simulink model "ACC5v_FFNN_traincgf_30_30_30_ep_50_Nor_20250704"  (R2021a)
settings: Solver=FixedStepAuto  StartTime=0.0  StopTime=T  RelTol=1e-3
undefined symbols (not defined in the file or in its folder): t_gap, Ts, v0_ego, v0_lead, v_set, x0_ego, x0_lead, x_gain, x_offset, y_gain, y_offset
libraries: neural x95
(part 1 of 5)
settings Model: Creator=The MathWorks, Inc.  LastModifiedBy=deyun
settings SolverCC: AlgebraicLoopSolver=TrustRegion
settings DataIOCC: ReturnWorkspaceOutputs=off
settings DebuggingCC: ArithmeticOperatorsInVariantConditions=warning
settings SFSimCC: SimUseLocalCustomCode=off  CustomCodeUndefinedFunction=UseInterfaceOnly
settings RTWCC: RTWUseLocalCustomCode=off
settings CodeAppCC: StateflowObjectComments=on

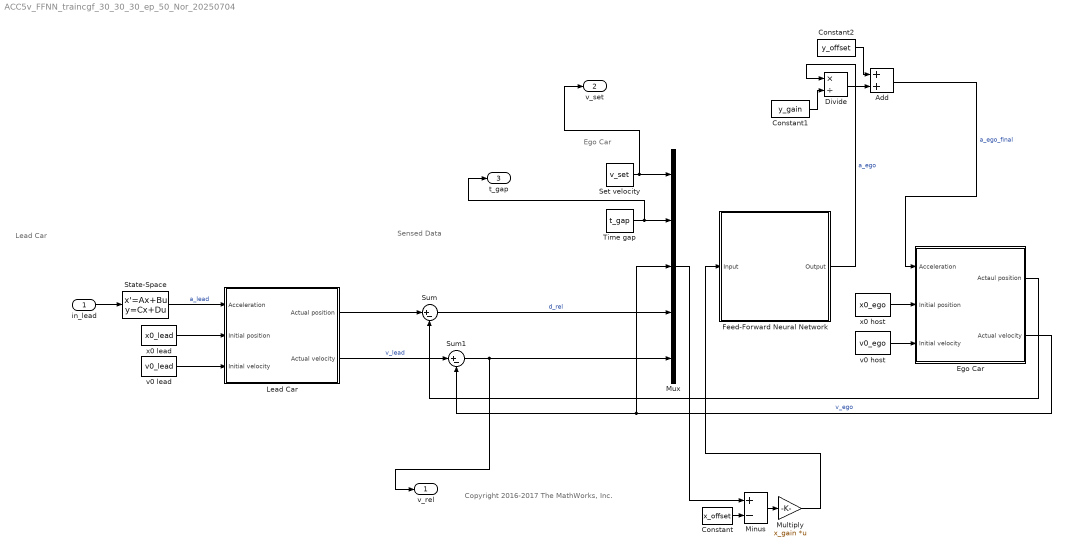
== system ACC5v_FFNN_traincgf_30_30_30_ep_50_Nor_20250704 ==
  note: Sensed Data
  note: Lead Car
  note: Ego Car
  note: Copyright 2016-2017 The MathWorks, Inc.
  in_lead : Inport
  Add : Sum
  Constant : Constant  Value=x_offset
  Constant1 : Constant  Value=y_gain
  Constant2 : Constant  Value=y_offset
  Divide : Product  Inputs=*/
  Ego Car : Subsystem
  Feed-Forward Neural Network : Subsystem
      mask help: Feed-Forward Neural Network
      mask Display: e = 0.06;c1 = [120 150 230]/255;c2 = ([120 150 230]+0)/383;c3 = ([120 150 230]+128)/383;patch([0 1 1 0],[0 0 1 1],c1);patch([0 1 1 1-e 1-e 0+e],[0 0 1 1-e 0+e 0+e],c2);patch([0 0 1 1-e 0+e 0+e],[0 1 1 1-e 1-e 0+e],c3);plot([0 1 1 0 0],[0 0 1 1 0]);fprintf('NNET');port_label('input',1,' Input');port_label('output',1,'Output ');
  Lead Car : Subsystem
  Minus : Sum  Inputs=+-
  Multiply : Gain  Gain=x_gain  Multiplication=Matrix(K*u)
  Mux : Mux  Inputs=5
  Set velocity : Constant  Value=v_set  SampleTime=Ts
  State-Space : StateSpace  A=-10  B=10  D=0  InitialCondition=0
  Sum : Sum  Inputs=|+-
  Sum1 : Sum  Inputs=|+-
  Time gap : Constant  Value=t_gap  SampleTime=Ts
  v0 host : Constant  Value=v0_ego  SampleTime=Ts
  v0 lead : Constant  Value=v0_lead  SampleTime=Ts
  x0 host : Constant  Value=x0_ego  SampleTime=Ts
  x0 lead : Constant  Value=x0_lead  SampleTime=Ts
  v_rel : Outport
  v_set : Outport  Port=2
  t_gap : Outport  Port=3
  wires:
  x0 lead/1 -> Lead Car/2(Initial position)
  v0 lead/1 -> Lead Car/3(Initial velocity)
  x0 host/1 -> Ego Car/2(Initial position)
  Ego Car/1(Actaul position) -> Sum/2
  Ego Car/2(Actual velocity) -> Mux/3, Sum1/2  "v_ego"
  v0 host/1 -> Ego Car/3(Initial velocity)
  Set velocity/1 -> v_set/1, Mux/1
  Feed-Forward Neural Network/1(Output) -> Divide/1  "a_ego"
  Lead Car/1(Actual position) -> Sum/1
  Sum1/1 -> v_rel/1, Mux/5
  State-Space/1 -> Lead Car/1(Acceleration)  "a_lead"
  Lead Car/2(Actual velocity) -> Sum1/1  "v_lead"
  Sum/1 -> Mux/4  "d_rel"
  in_lead/1 -> State-Space/1
  Time gap/1 -> t_gap/1, Mux/2
  Mux/1 -> Minus/1
  Minus/1 -> Multiply/1
  Constant/1 -> Minus/2
  Multiply/1 -> Feed-Forward Neural Network/1(Input)
  Constant1/1 -> Divide/2
  Divide/1 -> Add/2
  Constant2/1 -> Add/1
  Add/1 -> Ego Car/1(Acceleration)  "a_ego_final"

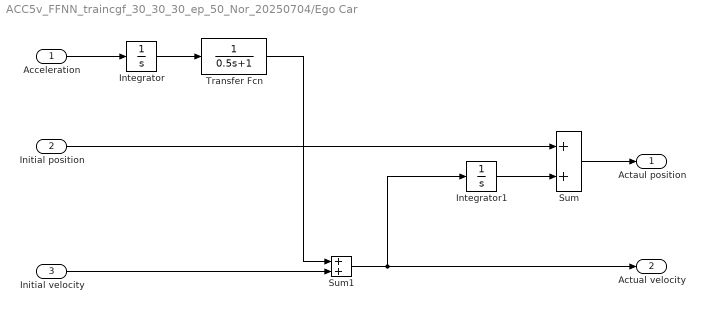
== system ACC5v_FFNN_traincgf_30_30_30_ep_50_Nor_20250704/Ego Car ==
  Acceleration : Inport
  Initial position : Inport  Port=2
  Initial velocity : Inport  Port=3
  Integrator : Integrator
  Integrator1 : Integrator
  Sum : Sum
  Sum1 : Sum
  Transfer Fcn : TransferFcn  Denominator=[0.5 1]
  Actaul position : Outport  VectorParamsAs1DForOutWhenUnconnected=off
  Actual velocity : Outport  Port=2  VectorParamsAs1DForOutWhenUnconnected=off
  wires:
  Sum1/1 -> Integrator1/1, Actual velocity/1
  Initial velocity/1 -> Sum1/2
  Sum/1 -> Actaul position/1
  Transfer Fcn/1 -> Sum1/1
  Integrator/1 -> Transfer Fcn/1
  Acceleration/1 -> Integrator/1
  Initial position/1 -> Sum/1
  Integrator1/1 -> Sum/2

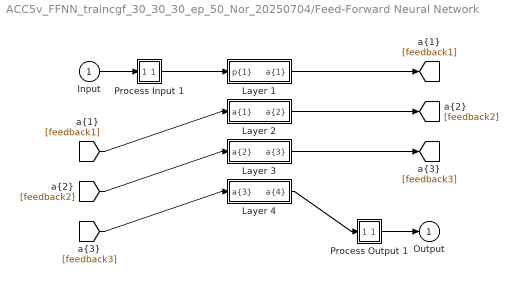
== system ACC5v_FFNN_traincgf_30_30_30_ep_50_Nor_20250704/Feed-Forward Neural Network ==
  Input : Inport  PortDimensions=5
      mask Display: e = 0.06;c1 = [120 230 180]/255;c2 = ([120 230 180]+0)/(256+128);c3 = ([120 230 180]+128)/(256+128);patch([0 1 1 0],[0 0 1 1],c1);patch([0 1 1 1-e 1-e 0+e],[0 0 1 1-e 0+e 0+e],c2);patch([0 0 1 1-e 0+e 0+e],[0 1 1 1-e 1-e 0+e],c3);plot([0 1 1 0 0],[0 0 1 1 0]);
  Layer 1 : Subsystem
      mask Display: e = 0.06;c1 = [120 150 230]/255;c2 = ([120 150 230]+0)/383;c3 = ([120 150 230]+128)/383;patch([0 1 1 0],[0 0 1 1],c1);patch([0 1 1 1-e 1-e 0+e],[0 0 1 1-e 0+e 0+e],c2);patch([0 0 1 1-e 0+e 0+e],[0 1 1 1-e 1-e 0+e],c3);plot([0 1 1 0 0],[0 0 1 1 0]);
  Layer 2 : Subsystem
      mask Display: e = 0.06;c1 = [120 150 230]/255;c2 = ([120 150 230]+0)/383;c3 = ([120 150 230]+128)/383;patch([0 1 1 0],[0 0 1 1],c1);patch([0 1 1 1-e 1-e 0+e],[0 0 1 1-e 0+e 0+e],c2);patch([0 0 1 1-e 0+e 0+e],[0 1 1 1-e 1-e 0+e],c3);plot([0 1 1 0 0],[0 0 1 1 0]);
  Layer 3 : Subsystem
      mask Display: e = 0.06;c1 = [120 150 230]/255;c2 = ([120 150 230]+0)/383;c3 = ([120 150 230]+128)/383;patch([0 1 1 0],[0 0 1 1],c1);patch([0 1 1 1-e 1-e 0+e],[0 0 1 1-e 0+e 0+e],c2);patch([0 0 1 1-e 0+e 0+e],[0 1 1 1-e 1-e 0+e],c3);plot([0 1 1 0 0],[0 0 1 1 0]);
  Layer 4 : Subsystem
      mask Display: e = 0.06;c1 = [120 150 230]/255;c2 = ([120 150 230]+0)/383;c3 = ([120 150 230]+128)/383;patch([0 1 1 0],[0 0 1 1],c1);patch([0 1 1 1-e 1-e 0+e],[0 0 1 1-e 0+e 0+e],c2);patch([0 0 1 1-e 0+e 0+e],[0 1 1 1-e 1-e 0+e],c3);plot([0 1 1 0 0],[0 0 1 1 0]);
  Process Input 1 : Subsystem
      mask Display: e = 0.06;c1 = [120 150 230]/255;c2 = ([120 150 230]+0)/383;c3 = ([120 150 230]+128)/383;patch([0 1 1 0],[0 0 1 1],c1);patch([0 1 1 1-e 1-e 0+e],[0 0 1 1-e 0+e 0+e],c2);patch([0 0 1 1-e 0+e 0+e],[0 1 1 1-e 1-e 0+e],c3);plot([0 1 1 0 0],[0 0 1 1 0]);
  Process Output 1 : Subsystem
      mask Display: e = 0.06;c1 = [120 150 230]/255;c2 = ([120 150 230]+0)/383;c3 = ([120 150 230]+128)/383;patch([0 1 1 0],[0 0 1 1],c1);patch([0 1 1 1-e 1-e 0+e],[0 0 1 1-e 0+e 0+e],c2);patch([0 0 1 1-e 0+e 0+e],[0 1 1 1-e 1-e 0+e],c3);plot([0 1 1 0 0],[0 0 1 1 0]);
  Output : Outport  InitialOutput=0
      mask Display: e = 0.06;c1 = [120 230 180]/255;c2 = ([120 230 180]+0)/(256+128);c3 = ([120 230 180]+128)/(256+128);patch([0 1 1 0],[0 0 1 1],c1);patch([0 1 1 1-e 1-e 0+e],[0 0 1 1-e 0+e 0+e],c2);patch([0 0 1 1-e 0+e 0+e],[0 1 1 1-e 1-e 0+e],c3);plot([0 1 1 0 0],[0 0 1 1 0]);
  wires:
  Layer 4/1("a{4}") -> Process Output 1/1(a)
  [feedback3] -> Layer 4/1("a{3} ")
  Layer 3/1("a{3}") -> [feedback3]
  [feedback2] -> Layer 3/1("a{2} ")
  Layer 2/1("a{2}") -> [feedback2]
  [feedback1] -> Layer 2/1("a{1} ")
  Layer 1/1("a{1}") -> [feedback1]
  Process Input 1/1(p) -> Layer 1/1("p{1}")
  Process Output 1/1(y) -> Output/1
  Input/1 -> Process Input 1/1(x)

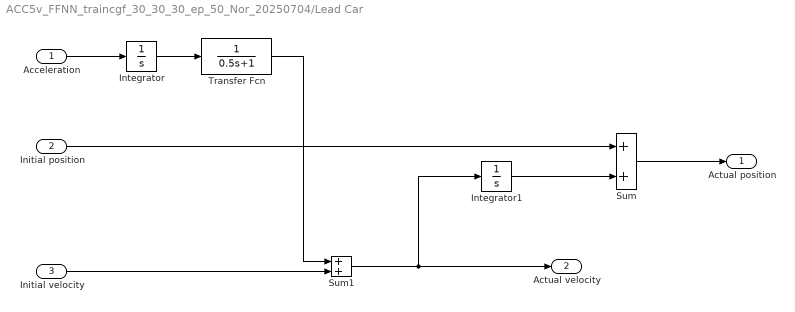
== system ACC5v_FFNN_traincgf_30_30_30_ep_50_Nor_20250704/Lead Car ==
  Acceleration : Inport
  Initial position : Inport  Port=2
  Initial velocity : Inport  Port=3
  Integrator : Integrator
  Integrator1 : Integrator
  Sum : Sum
  Sum1 : Sum
  Transfer Fcn : TransferFcn  Denominator=[0.5 1]
  Actual position : Outport  VectorParamsAs1DForOutWhenUnconnected=off
  Actual velocity : Outport  Port=2  VectorParamsAs1DForOutWhenUnconnected=off
  wires:
  Transfer Fcn/1 -> Sum1/1
  Initial velocity/1 -> Sum1/2
  Sum/1 -> Actual position/1
  Integrator/1 -> Transfer Fcn/1
  Sum1/1 -> Integrator1/1, Actual velocity/1
  Acceleration/1 -> Integrator/1
  Initial position/1 -> Sum/1
  Integrator1/1 -> Sum/2

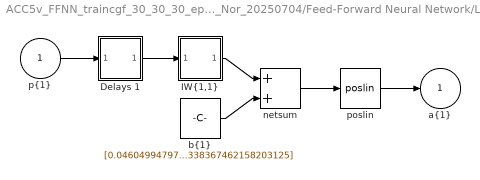
== system ACC5v_FFNN_traincgf_30_30_30_ep_50_Nor_20250704/Feed-Forward Neural Network/Layer 1 ==
  "p{1}" : Inport  PortDimensions=5
      mask Display: e = 0.06;c1 = [120 230 180]/255;c2 = ([120 230 180]+0)/(256+128);c3 = ([120 230 180]+128)/(256+128);patch([0 1 1 0],[0 0 1 1],c1);patch([0 1 1 1-e 1-e 0+e],[0 0 1 1-e 0+e 0+e],c2);patch([0 0 1 1-e 0+e 0+e],[0 1 1 1-e 1-e 0+e],c3);plot([0 1 1 0 0],[0 0 1 1 0]);
  Delays 1 : Subsystem
      mask Display: e = 0.06;c1 = [120 150 230]/255;c2 = ([120 150 230]+0)/383;c3 = ([120 150 230]+128)/383;patch([0 1 1 0],[0 0 1 1],c1);patch([0 1 1 1-e 1-e 0+e],[0 0 1 1-e 0+e 0+e],c2);patch([0 0 1 1-e 0+e 0+e],[0 1 1 1-e 1-e 0+e],c3);plot([0 1 1 0 0],[0 0 1 1 0]);disp('0');
  "IW{1,1}" : Subsystem
      mask Display: e = 0.06;c1 = [120 150 230]/255;c2 = ([120 150 230]+0)/383;c3 = ([120 150 230]+128)/383;patch([0 1 1 0],[0 0 1 1],c1);patch([0 1 1 1-e 1-e 0+e],[0 0 1 1-e 0+e 0+e],c2);patch([0 0 1 1-e 0+e 0+e],[0 1 1 1-e 1-e 0+e],c3);plot([0 1 1 0 0],[0 0 1 1 0]);disp('W');
  "b{1}" : Constant  Value=[0.0460499479730639149632764883790514431893825531005859375;-0.349402015011147870637842061114497482776641845703125;0.66507025600709568369239832463790662586688995361328125;0.60741250780027267186511608088039793074131011962890625;0.126284847005241951389820087570114992558956146240234375;-0.4740719325396856032028836125391535460948944091796875;0.3611324046089003925175120457424782216548919677734375;-0.5319955567783940519888119524694047868251800537109375;-0.08710031213979936570712681032091495580971240997314453125;-0.230866210976952146438634372316300868988037109375;0.077202877396043589897089987061917781829833984375;1.0025558120245303683759630075655877590179443359375;0.497318027802917728141807174324640072882175445556640625;0.9553277572718903432047454771236516535282135009765625;-0.496332469052459479552652510392363183200359344482421875;0.045748943680550525903161229734905646182596683502197265625;-0.897127892866184328823919713613577187061309814453125;0.5137509419692445344907127946498803794384002685546875;0.20395953255102039491930554504506289958953857421875;0.708157197743781718912714495672844350337982177734375;0.9532103730466758850781161527265794575214385986328125;0.85600360045154000321332432577037252485752105712890625;-0.165015832658127525878200003717211075127124786376953125;-1.004030844730705585021723891259171068668365478515625;0.0873034903187444033534347909153439104557037353515625;-0.5845387560078811883812477390165440738201141357421875;-0.5614328236351393552894251115503720939159393310546875;-0.3537174892029881778654498702962882816791534423828125;-0.80810116678483101537722177454270422458648681640625;0.4950673234766060915035268408246338367462158203125]
      mask Display: e = 0.06;c1 = [120 150 230]/255;c2 = ([120 150 230]+0)/383;c3 = ([120 150 230]+128)/383;patch([0 1 1 0],[0 0 1 1],c1);patch([0 1 1 1-e 1-e 0+e],[0 0 1 1-e 0+e 0+e],c2);patch([0 0 1 1-e 0+e 0+e],[0 1 1 1-e 1-e 0+e],c3);plot([0 1 1 0 0],[0 0 1 1 0]);disp('b');
  netsum : Sum  Inputs=2  InputSameDT=on  SaturateOnIntegerOverflow=on  OutDataTypeStr=Inherit: Same as first input
      mask Display: e = 0.06;c1 = [120 150 230]/255;c2 = ([120 150 230]+0)/383;c3 = ([120 150 230]+128)/383;patch([0 1 1 0],[0 0 1 1],c1);patch([0 1 1 1-e 1-e 0+e],[0 0 1 1-e 0+e 0+e],c2);patch([0 0 1 1-e 0+e 0+e],[0 1 1 1-e 1-e 0+e],c3);plot([0 1 1 0 0],[0 0 1 1 0]);disp('+');
  poslin : neural/Transfer Functions/poslin
      settings: SourceProductBaseCode=NN
  "a{1}" : Outport  InitialOutput=[0;0;0;0;0;0;0;0;0;0;0;0;0;0;0;0;0;0;0;0;0;0;0;0;0;0;0;0;0;0]
      mask Display: e = 0.06;c1 = [120 230 180]/255;c2 = ([120 230 180]+0)/(256+128);c3 = ([120 230 180]+128)/(256+128);patch([0 1 1 0],[0 0 1 1],c1);patch([0 1 1 1-e 1-e 0+e],[0 0 1 1-e 0+e 0+e],c2);patch([0 0 1 1-e 0+e 0+e],[0 1 1 1-e 1-e 0+e],c3);plot([0 1 1 0 0],[0 0 1 1 0]);
  wires:
  poslin/1 -> "a{1}"/1
  netsum/1 -> poslin/1
  "b{1}"/1 -> netsum/2
  "IW{1,1}"/1("iz{1,1}") -> netsum/1
  Delays 1/1("pd{1,1}") -> "IW{1,1}"/1("pd{1,1}")
  "p{1}"/1 -> Delays 1/1("p{1}")

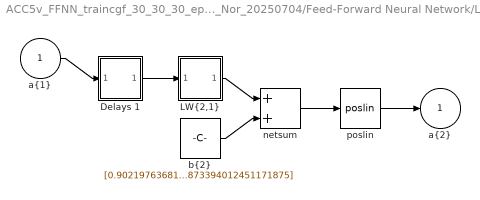
== system ACC5v_FFNN_traincgf_30_30_30_ep_50_Nor_20250704/Feed-Forward Neural Network/Layer 2 ==
  "a{1} " : Inport  PortDimensions=30
      mask Display: e = 0.06;c1 = [120 230 180]/255;c2 = ([120 230 180]+0)/(256+128);c3 = ([120 230 180]+128)/(256+128);patch([0 1 1 0],[0 0 1 1],c1);patch([0 1 1 1-e 1-e 0+e],[0 0 1 1-e 0+e 0+e],c2);patch([0 0 1 1-e 0+e 0+e],[0 1 1 1-e 1-e 0+e],c3);plot([0 1 1 0 0],[0 0 1 1 0]);
  Delays 1 : Subsystem
      mask Display: e = 0.06;c1 = [120 150 230]/255;c2 = ([120 150 230]+0)/383;c3 = ([120 150 230]+128)/383;patch([0 1 1 0],[0 0 1 1],c1);patch([0 1 1 1-e 1-e 0+e],[0 0 1 1-e 0+e 0+e],c2);patch([0 0 1 1-e 0+e 0+e],[0 1 1 1-e 1-e 0+e],c3);plot([0 1 1 0 0],[0 0 1 1 0]);disp('0');
  "LW{2,1}" : Subsystem
      mask Display: e = 0.06;c1 = [120 150 230]/255;c2 = ([120 150 230]+0)/383;c3 = ([120 150 230]+128)/383;patch([0 1 1 0],[0 0 1 1],c1);patch([0 1 1 1-e 1-e 0+e],[0 0 1 1-e 0+e 0+e],c2);patch([0 0 1 1-e 0+e 0+e],[0 1 1 1-e 1-e 0+e],c3);plot([0 1 1 0 0],[0 0 1 1 0]);disp('W');
  "b{2}" : Constant  Value=[0.9021976368187230033157675279653631150722503662109375;0.96422796298322588359752671749447472393512725830078125;-0.93804589522122638900469837608397938311100006103515625;-0.01535281312125513254740472035564380348660051822662353515625;0.725444256277659516030098529881797730922698974609375;-0.511127433954644327940286530065350234508514404296875;0.6651683692220642374337558067054487764835357666015625;0.62723629167634797898500664814491756260395050048828125;0.25901176430492045543729773271479643881320953369140625;-0.9939790090024456237216554654878564178943634033203125;-0.2405521205461311762263676428119651973247528076171875;0.80883631394758737087613553740084171295166015625;0.360880159162838942688011911741341464221477508544921875;-0.2430011681204506668318998663380625657737255096435546875;0.2639094214046682207452931834268383681774139404296875;-0.5134609550588200566068053376511670649051666259765625;0.1363991749822880683584713779055164195597171783447265625;0.97850079917507304383406108172493986785411834716796875;0.6950934096731484768127984352759085595607757568359375;-0.435098409889481840817637703366926871240139007568359375;0.364915328900436097825377146364189684391021728515625;-0.279181296811478574237952443581889383494853973388671875;0.97801571639253637169275634732912294566631317138671875;-0.832027408487622466282118693925440311431884765625;-0.49363837291945877883136972741340287029743194580078125;0.6267534454383854036763068506843410432338714599609375;-0.83097531923572354184415189592982642352581024169921875;0.06341854724127198028593710432687657885253429412841796875;0.601245958295900440049308599554933607578277587890625;0.478255302509084045947673757837037555873394012451171875]
      mask Display: e = 0.06;c1 = [120 150 230]/255;c2 = ([120 150 230]+0)/383;c3 = ([120 150 230]+128)/383;patch([0 1 1 0],[0 0 1 1],c1);patch([0 1 1 1-e 1-e 0+e],[0 0 1 1-e 0+e 0+e],c2);patch([0 0 1 1-e 0+e 0+e],[0 1 1 1-e 1-e 0+e],c3);plot([0 1 1 0 0],[0 0 1 1 0]);disp('b');
  netsum : Sum  Inputs=2  InputSameDT=on  SaturateOnIntegerOverflow=on  OutDataTypeStr=Inherit: Same as first input
      mask Display: e = 0.06;c1 = [120 150 230]/255;c2 = ([120 150 230]+0)/383;c3 = ([120 150 230]+128)/383;patch([0 1 1 0],[0 0 1 1],c1);patch([0 1 1 1-e 1-e 0+e],[0 0 1 1-e 0+e 0+e],c2);patch([0 0 1 1-e 0+e 0+e],[0 1 1 1-e 1-e 0+e],c3);plot([0 1 1 0 0],[0 0 1 1 0]);disp('+');
  poslin : neural/Transfer Functions/poslin
      settings: SourceProductBaseCode=NN
  "a{2}" : Outport  InitialOutput=[0;0;0;0;0;0;0;0;0;0;0;0;0;0;0;0;0;0;0;0;0;0;0;0;0;0;0;0;0;0]
      mask Display: e = 0.06;c1 = [120 230 180]/255;c2 = ([120 230 180]+0)/(256+128);c3 = ([120 230 180]+128)/(256+128);patch([0 1 1 0],[0 0 1 1],c1);patch([0 1 1 1-e 1-e 0+e],[0 0 1 1-e 0+e 0+e],c2);patch([0 0 1 1-e 0+e 0+e],[0 1 1 1-e 1-e 0+e],c3);plot([0 1 1 0 0],[0 0 1 1 0]);
  wires:
  poslin/1 -> "a{2}"/1
  netsum/1 -> poslin/1
  "b{2}"/1 -> netsum/2
  "LW{2,1}"/1("lz{2,1}") -> netsum/1
  Delays 1/1("pd{2,1}") -> "LW{2,1}"/1("ad{2,1}")
  "a{1} "/1 -> Delays 1/1("p{2}")

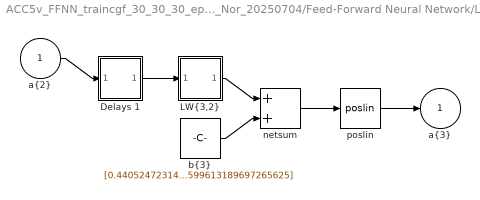
== system ACC5v_FFNN_traincgf_30_30_30_ep_50_Nor_20250704/Feed-Forward Neural Network/Layer 3 ==
  "a{2} " : Inport  PortDimensions=30
      mask Display: e = 0.06;c1 = [120 230 180]/255;c2 = ([120 230 180]+0)/(256+128);c3 = ([120 230 180]+128)/(256+128);patch([0 1 1 0],[0 0 1 1],c1);patch([0 1 1 1-e 1-e 0+e],[0 0 1 1-e 0+e 0+e],c2);patch([0 0 1 1-e 0+e 0+e],[0 1 1 1-e 1-e 0+e],c3);plot([0 1 1 0 0],[0 0 1 1 0]);
  Delays 1 : Subsystem
      mask Display: e = 0.06;c1 = [120 150 230]/255;c2 = ([120 150 230]+0)/383;c3 = ([120 150 230]+128)/383;patch([0 1 1 0],[0 0 1 1],c1);patch([0 1 1 1-e 1-e 0+e],[0 0 1 1-e 0+e 0+e],c2);patch([0 0 1 1-e 0+e 0+e],[0 1 1 1-e 1-e 0+e],c3);plot([0 1 1 0 0],[0 0 1 1 0]);disp('0');
  "LW{3,2}" : Subsystem
      mask Display: e = 0.06;c1 = [120 150 230]/255;c2 = ([120 150 230]+0)/383;c3 = ([120 150 230]+128)/383;patch([0 1 1 0],[0 0 1 1],c1);patch([0 1 1 1-e 1-e 0+e],[0 0 1 1-e 0+e 0+e],c2);patch([0 0 1 1-e 0+e 0+e],[0 1 1 1-e 1-e 0+e],c3);plot([0 1 1 0 0],[0 0 1 1 0]);disp('W');
  "b{3}" : Constant  Value=[0.4405247231410467367851424569380469620227813720703125;0.357972491709714624175120434301788918673992156982421875;-0.574481979793593833250042735016904771327972412109375;-0.8372018435998034302514270166284404695034027099609375;-0.451475326916109420682943209612858481705188751220703125;0.73636285635996656662172199503402225673198699951171875;0.1183228140510626802406335400519310496747493743896484375;-0.07103643217944512200379136857009143568575382232666015625;-0.1393981984391927664290733446250669658184051513671875;0.54797184004082755137687854585237801074981689453125;0.308391888747984344032460057860589586198329925537109375;0.3154544543298969383471330729662440717220306396484375;-0.67805761599920078008807422520476393401622772216796875;-0.1352516737627559584300485084895626641809940338134765625;0.010172168711043649835801261360757052898406982421875;-0.253953321988893920835295148208388127386569976806640625;-0.039775072451052113919889308135680039413273334503173828125;-0.31526147340369214955302368252887390553951263427734375;0.5551748462880412571252009001909755170345306396484375;-0.2321122752203861328013090314925648272037506103515625;0.4234595840265191757367801983491517603397369384765625;-0.040296552567531007671419729376793839037418365478515625;0.45836044424314348333382440614514052867889404296875;0.8749079983785374992066863342188298702239990234375;0.034027996391464747361066400799245457164943218231201171875;0.80613117416423507588518759803264401853084564208984375;-0.56321446665910401829790998817770741879940032958984375;0.74661057287508214574955900388886220753192901611328125;-0.8343441643403217700125651390408165752887725830078125;-0.0690161403682808816117955075242207385599613189697265625]
      mask Display: e = 0.06;c1 = [120 150 230]/255;c2 = ([120 150 230]+0)/383;c3 = ([120 150 230]+128)/383;patch([0 1 1 0],[0 0 1 1],c1);patch([0 1 1 1-e 1-e 0+e],[0 0 1 1-e 0+e 0+e],c2);patch([0 0 1 1-e 0+e 0+e],[0 1 1 1-e 1-e 0+e],c3);plot([0 1 1 0 0],[0 0 1 1 0]);disp('b');
  netsum : Sum  Inputs=2  InputSameDT=on  SaturateOnIntegerOverflow=on  OutDataTypeStr=Inherit: Same as first input
      mask Display: e = 0.06;c1 = [120 150 230]/255;c2 = ([120 150 230]+0)/383;c3 = ([120 150 230]+128)/383;patch([0 1 1 0],[0 0 1 1],c1);patch([0 1 1 1-e 1-e 0+e],[0 0 1 1-e 0+e 0+e],c2);patch([0 0 1 1-e 0+e 0+e],[0 1 1 1-e 1-e 0+e],c3);plot([0 1 1 0 0],[0 0 1 1 0]);disp('+');
  poslin : neural/Transfer Functions/poslin
      settings: SourceProductBaseCode=NN
  "a{3}" : Outport  InitialOutput=[0;0;0;0;0;0;0;0;0;0;0;0;0;0;0;0;0;0;0;0;0;0;0;0;0;0;0;0;0;0]
      mask Display: e = 0.06;c1 = [120 230 180]/255;c2 = ([120 230 180]+0)/(256+128);c3 = ([120 230 180]+128)/(256+128);patch([0 1 1 0],[0 0 1 1],c1);patch([0 1 1 1-e 1-e 0+e],[0 0 1 1-e 0+e 0+e],c2);patch([0 0 1 1-e 0+e 0+e],[0 1 1 1-e 1-e 0+e],c3);plot([0 1 1 0 0],[0 0 1 1 0]);
  wires:
  poslin/1 -> "a{3}"/1
  netsum/1 -> poslin/1
  "b{3}"/1 -> netsum/2
  "LW{3,2}"/1("lz{3,2}") -> netsum/1
  Delays 1/1("pd{3,2}") -> "LW{3,2}"/1("ad{3,2}")
  "a{2} "/1 -> Delays 1/1("p{3}")

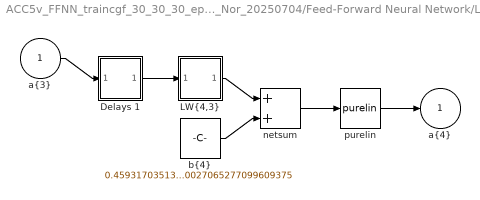
== system ACC5v_FFNN_traincgf_30_30_30_ep_50_Nor_20250704/Feed-Forward Neural Network/Layer 4 ==
  "a{3} " : Inport  PortDimensions=30
      mask Display: e = 0.06;c1 = [120 230 180]/255;c2 = ([120 230 180]+0)/(256+128);c3 = ([120 230 180]+128)/(256+128);patch([0 1 1 0],[0 0 1 1],c1);patch([0 1 1 1-e 1-e 0+e],[0 0 1 1-e 0+e 0+e],c2);patch([0 0 1 1-e 0+e 0+e],[0 1 1 1-e 1-e 0+e],c3);plot([0 1 1 0 0],[0 0 1 1 0]);
  Delays 1 : Subsystem
      mask Display: e = 0.06;c1 = [120 150 230]/255;c2 = ([120 150 230]+0)/383;c3 = ([120 150 230]+128)/383;patch([0 1 1 0],[0 0 1 1],c1);patch([0 1 1 1-e 1-e 0+e],[0 0 1 1-e 0+e 0+e],c2);patch([0 0 1 1-e 0+e 0+e],[0 1 1 1-e 1-e 0+e],c3);plot([0 1 1 0 0],[0 0 1 1 0]);disp('0');
  "LW{4,3}" : Subsystem
      mask Display: e = 0.06;c1 = [120 150 230]/255;c2 = ([120 150 230]+0)/383;c3 = ([120 150 230]+128)/383;patch([0 1 1 0],[0 0 1 1],c1);patch([0 1 1 1-e 1-e 0+e],[0 0 1 1-e 0+e 0+e],c2);patch([0 0 1 1-e 0+e 0+e],[0 1 1 1-e 1-e 0+e],c3);plot([0 1 1 0 0],[0 0 1 1 0]);disp('W');
  "b{4}" : Constant  Value=0.45931703513931443350060135344392620027065277099609375
      mask Display: e = 0.06;c1 = [120 150 230]/255;c2 = ([120 150 230]+0)/383;c3 = ([120 150 230]+128)/383;patch([0 1 1 0],[0 0 1 1],c1);patch([0 1 1 1-e 1-e 0+e],[0 0 1 1-e 0+e 0+e],c2);patch([0 0 1 1-e 0+e 0+e],[0 1 1 1-e 1-e 0+e],c3);plot([0 1 1 0 0],[0 0 1 1 0]);disp('b');
  netsum : Sum  Inputs=2  InputSameDT=on  SaturateOnIntegerOverflow=on  OutDataTypeStr=Inherit: Same as first input
      mask Display: e = 0.06;c1 = [120 150 230]/255;c2 = ([120 150 230]+0)/383;c3 = ([120 150 230]+128)/383;patch([0 1 1 0],[0 0 1 1],c1);patch([0 1 1 1-e 1-e 0+e],[0 0 1 1-e 0+e 0+e],c2);patch([0 0 1 1-e 0+e 0+e],[0 1 1 1-e 1-e 0+e],c3);plot([0 1 1 0 0],[0 0 1 1 0]);disp('+');
  purelin : neural/Transfer Functions/purelin
  "a{4}" : Outport  InitialOutput=0
      mask Display: e = 0.06;c1 = [120 230 180]/255;c2 = ([120 230 180]+0)/(256+128);c3 = ([120 230 180]+128)/(256+128);patch([0 1 1 0],[0 0 1 1],c1);patch([0 1 1 1-e 1-e 0+e],[0 0 1 1-e 0+e 0+e],c2);patch([0 0 1 1-e 0+e 0+e],[0 1 1 1-e 1-e 0+e],c3);plot([0 1 1 0 0],[0 0 1 1 0]);
  wires:
  purelin/1 -> "a{4}"/1
  netsum/1 -> purelin/1
  "b{4}"/1 -> netsum/2
  "LW{4,3}"/1("lz{4,3}") -> netsum/1
  Delays 1/1("pd{4,3}") -> "LW{4,3}"/1("ad{4,3}")
  "a{3} "/1 -> Delays 1/1("p{4}")

== system ACC5v_FFNN_traincgf_30_30_30_ep_50_Nor_20250704/Feed-Forward Neural Network/Process Input 1 ==
  x : Inport  PortDimensions=5
      mask Display: e = 0.06;c1 = [120 230 180]/255;c2 = ([120 230 180]+0)/(256+128);c3 = ([120 230 180]+128)/(256+128);patch([0 1 1 0],[0 0 1 1],c1);patch([0 1 1 1-e 1-e 0+e],[0 0 1 1-e 0+e 0+e],c2);patch([0 0 1 1-e 0+e 0+e],[0 1 1 1-e 1-e 0+e],c3);plot([0 1 1 0 0],[0 0 1 1 0]);
  p : Outport  PortDimensions=5
      mask Display: e = 0.06;c1 = [120 230 180]/255;c2 = ([120 230 180]+0)/(256+128);c3 = ([120 230 180]+128)/(256+128);patch([0 1 1 0],[0 0 1 1],c1);patch([0 1 1 1-e 1-e 0+e],[0 0 1 1-e 0+e 0+e],c2);patch([0 0 1 1-e 0+e 0+e],[0 1 1 1-e 1-e 0+e],c3);plot([0 1 1 0 0],[0 0 1 1 0]);
  wires:
  x/1 -> p/1

== system ACC5v_FFNN_traincgf_30_30_30_ep_50_Nor_20250704/Feed-Forward Neural Network/Process Output 1 ==
  a : Inport  PortDimensions=1
      mask Display: e = 0.06;c1 = [120 230 180]/255;c2 = ([120 230 180]+0)/(256+128);c3 = ([120 230 180]+128)/(256+128);patch([0 1 1 0],[0 0 1 1],c1);patch([0 1 1 1-e 1-e 0+e],[0 0 1 1-e 0+e 0+e],c2);patch([0 0 1 1-e 0+e 0+e],[0 1 1 1-e 1-e 0+e],c3);plot([0 1 1 0 0],[0 0 1 1 0]);
  y : Outport  PortDimensions=1
      mask Display: e = 0.06;c1 = [120 230 180]/255;c2 = ([120 230 180]+0)/(256+128);c3 = ([120 230 180]+128)/(256+128);patch([0 1 1 0],[0 0 1 1],c1);patch([0 1 1 1-e 1-e 0+e],[0 0 1 1-e 0+e 0+e],c2);patch([0 0 1 1-e 0+e 0+e],[0 1 1 1-e 1-e 0+e],c3);plot([0 1 1 0 0],[0 0 1 1 0]);
  wires:
  a/1 -> y/1

== system ACC5v_FFNN_traincgf_30_30_30_ep_50_Nor_20250704/Feed-Forward Neural Network/Layer 1/Delays 1 ==
  "p{1}" : Inport  PortDimensions=5
      mask Display: e = 0.06;c1 = [120 230 180]/255;c2 = ([120 230 180]+0)/(256+128);c3 = ([120 230 180]+128)/(256+128);patch([0 1 1 0],[0 0 1 1],c1);patch([0 1 1 1-e 1-e 0+e],[0 0 1 1-e 0+e 0+e],c2);patch([0 0 1 1-e 0+e 0+e],[0 1 1 1-e 1-e 0+e],c3);plot([0 1 1 0 0],[0 0 1 1 0]);
  mux : Mux  Inputs=1
      mask Display: e = 0.06;c1 = [120 150 230]/255;c2 = ([120 150 230]+0)/383;c3 = ([120 150 230]+128)/383;patch([0 1 1 0],[0 0 1 1],c1);patch([0 1 1 1-e 1-e 0+e],[0 0 1 1-e 0+e 0+e],c2);patch([0 0 1 1-e 0+e 0+e],[0 1 1 1-e 1-e 0+e],c3);plot([0 1 1 0 0],[0 0 1 1 0]);disp('Mux')
  "pd{1,1}" : Outport
      mask Display: e = 0.06;c1 = [120 230 180]/255;c2 = ([120 230 180]+0)/(256+128);c3 = ([120 230 180]+128)/(256+128);patch([0 1 1 0],[0 0 1 1],c1);patch([0 1 1 1-e 1-e 0+e],[0 0 1 1-e 0+e 0+e],c2);patch([0 0 1 1-e 0+e 0+e],[0 1 1 1-e 1-e 0+e],c3);plot([0 1 1 0 0],[0 0 1 1 0]);
  wires:
  mux/1 -> "pd{1,1}"/1
  "p{1}"/1 -> mux/1

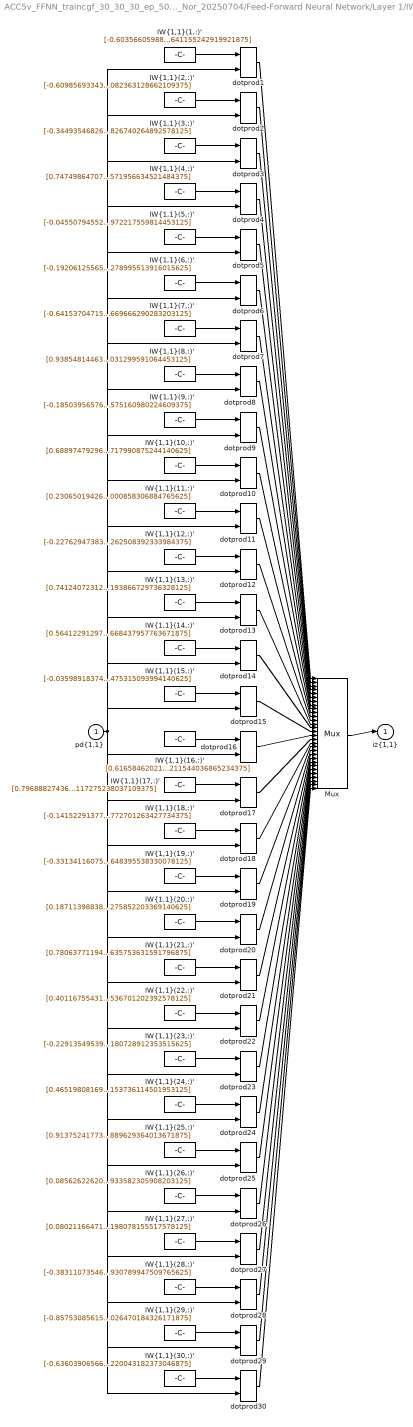
== system ACC5v_FFNN_traincgf_30_30_30_ep_50_Nor_20250704/Feed-Forward Neural Network/Layer 1/IW{1,1} ==
  "pd{1,1}" : Inport  PortDimensions=5
      mask Display: e = 0.06;c1 = [120 230 180]/255;c2 = ([120 230 180]+0)/(256+128);c3 = ([120 230 180]+128)/(256+128);patch([0 1 1 0],[0 0 1 1],c1);patch([0 1 1 1-e 1-e 0+e],[0 0 1 1-e 0+e 0+e],c2);patch([0 0 1 1-e 0+e 0+e],[0 1 1 1-e 1-e 0+e],c3);plot([0 1 1 0 0],[0 0 1 1 0]);
  "IW{1,1}(1,:)'" : Constant  Value=[-0.6035660598832441881000931971357204020023345947265625;-0.814031795169566141368022726965136826038360595703125;-0.07754612792111857666466079308520420454442501068115234375;0.71378313244740632104168298610602505505084991455078125;0.790837427247744084723990454222075641155242919921875]
      mask Display: e = 0.06;c1 = [120 150 230]/255;c2 = ([120 150 230]+0)/383;c3 = ([120 150 230]+128)/383;patch([0 1 1 0],[0 0 1 1],c1);patch([0 1 1 1-e 1-e 0+e],[0 0 1 1-e 0+e 0+e],c2);patch([0 0 1 1-e 0+e 0+e],[0 1 1 1-e 1-e 0+e],c3);plot([0 1 1 0 0],[0 0 1 1 0]);disp('Weights');
  "IW{1,1}(10,:)'" : Constant  Value=[0.6889747929668963433158523912425152957439422607421875;-0.745467933349733158365779672749340534210205078125;-0.64204969474453577049644081853330135345458984375;0.799965592865721664139755375799722969532012939453125;-0.6903424584977886357961551766493357717990875244140625]
      mask Display: e = 0.06;c1 = [120 150 230]/255;c2 = ([120 150 230]+0)/383;c3 = ([120 150 230]+128)/383;patch([0 1 1 0],[0 0 1 1],c1);patch([0 1 1 1-e 1-e 0+e],[0 0 1 1-e 0+e 0+e],c2);patch([0 0 1 1-e 0+e 0+e],[0 1 1 1-e 1-e 0+e],c3);plot([0 1 1 0 0],[0 0 1 1 0]);disp('Weights');
  "IW{1,1}(11,:)'" : Constant  Value=[0.230650194261698970876750536262989044189453125;-0.982704624243819324647120083682239055633544921875;0.2666671606402430949600557141820900142192840576171875;-0.6131324961218160840559221469447948038578033447265625;-0.71218334265026417284616400138475000858306884765625]
      mask Display: e = 0.06;c1 = [120 150 230]/255;c2 = ([120 150 230]+0)/383;c3 = ([120 150 230]+128)/383;patch([0 1 1 0],[0 0 1 1],c1);patch([0 1 1 1-e 1-e 0+e],[0 0 1 1-e 0+e 0+e],c2);patch([0 0 1 1-e 0+e 0+e],[0 1 1 1-e 1-e 0+e],c3);plot([0 1 1 0 0],[0 0 1 1 0]);disp('Weights');
  "IW{1,1}(12,:)'" : Constant  Value=[-0.2276294738339056655807013385128811933100223541259765625;0.473307572397674458652971907213213853538036346435546875;0.264314907242817198618212159999529831111431121826171875;0.50200206247308531981587975678849034011363983154296875;0.210940844195459165089090447509079240262508392333984375]
      mask Display: e = 0.06;c1 = [120 150 230]/255;c2 = ([120 150 230]+0)/383;c3 = ([120 150 230]+128)/383;patch([0 1 1 0],[0 0 1 1],c1);patch([0 1 1 1-e 1-e 0+e],[0 0 1 1-e 0+e 0+e],c2);patch([0 0 1 1-e 0+e 0+e],[0 1 1 1-e 1-e 0+e],c3);plot([0 1 1 0 0],[0 0 1 1 0]);disp('Weights');
  "IW{1,1}(13,:)'" : Constant  Value=[0.74124072312145206087308224596199579536914825439453125;-0.304889843439569874217198730548261664807796478271484375;-0.352433525234456201946642295297351665794849395751953125;-0.302467218032611173672563609216012991964817047119140625;-0.489815895402557988091984952916391193866729736328125]
      mask Display: e = 0.06;c1 = [120 150 230]/255;c2 = ([120 150 230]+0)/383;c3 = ([120 150 230]+128)/383;patch([0 1 1 0],[0 0 1 1],c1);patch([0 1 1 1-e 1-e 0+e],[0 0 1 1-e 0+e 0+e],c2);patch([0 0 1 1-e 0+e 0+e],[0 1 1 1-e 1-e 0+e],c3);plot([0 1 1 0 0],[0 0 1 1 0]);disp('Weights');
  "IW{1,1}(14,:)'" : Constant  Value=[0.5641229129771894168499102306668646633625030517578125;0.5553099506031913268344624157180078327655792236328125;0.605705597185387301095715884002856910228729248046875;-0.16429594586990703408702074739267118275165557861328125;-0.350768197842642848183203341250191442668437957763671875]
      mask Display: e = 0.06;c1 = [120 150 230]/255;c2 = ([120 150 230]+0)/383;c3 = ([120 150 230]+128)/383;patch([0 1 1 0],[0 0 1 1],c1);patch([0 1 1 1-e 1-e 0+e],[0 0 1 1-e 0+e 0+e],c2);patch([0 0 1 1-e 0+e 0+e],[0 1 1 1-e 1-e 0+e],c3);plot([0 1 1 0 0],[0 0 1 1 0]);disp('Weights');
  "IW{1,1}(15,:)'" : Constant  Value=[-0.035989183749086627039925900817252113483846187591552734375;-0.0925844671075728431475226898328401148319244384765625;1.031427676530551895694998165708966553211212158203125;-0.698372538034429002351544113480485975742340087890625;-0.1847988777670043492040719002034165896475315093994140625]
      mask Display: e = 0.06;c1 = [120 150 230]/255;c2 = ([120 150 230]+0)/383;c3 = ([120 150 230]+128)/383;patch([0 1 1 0],[0 0 1 1],c1);patch([0 1 1 1-e 1-e 0+e],[0 0 1 1-e 0+e 0+e],c2);patch([0 0 1 1-e 0+e 0+e],[0 1 1 1-e 1-e 0+e],c3);plot([0 1 1 0 0],[0 0 1 1 0]);disp('Weights');
  "IW{1,1}(16,:)'" : Constant  Value=[0.61658462021708848599388375077978707849979400634765625;-0.1382596686802428920248786425872822292149066925048828125;0.95628273494270532584238253548392094671726226806640625;0.62138667655375456888577900826930999755859375;-0.197067508450964490318568778093322180211544036865234375]
      mask Display: e = 0.06;c1 = [120 150 230]/255;c2 = ([120 150 230]+0)/383;c3 = ([120 150 230]+128)/383;patch([0 1 1 0],[0 0 1 1],c1);patch([0 1 1 1-e 1-e 0+e],[0 0 1 1-e 0+e 0+e],c2);patch([0 0 1 1-e 0+e 0+e],[0 1 1 1-e 1-e 0+e],c3);plot([0 1 1 0 0],[0 0 1 1 0]);disp('Weights');
  "IW{1,1}(17,:)'" : Constant  Value=[0.796888274360240789206955014378763735294342041015625;-0.901573639287027273070407318300567567348480224609375;-0.7459261156102858780769793156650848686695098876953125;0.24984705569255449830734505667351186275482177734375;-0.2276177228781752770458979284740053117275238037109375]
      mask Display: e = 0.06;c1 = [120 150 230]/255;c2 = ([120 150 230]+0)/383;c3 = ([120 150 230]+128)/383;patch([0 1 1 0],[0 0 1 1],c1);patch([0 1 1 1-e 1-e 0+e],[0 0 1 1-e 0+e 0+e],c2);patch([0 0 1 1-e 0+e 0+e],[0 1 1 1-e 1-e 0+e],c3);plot([0 1 1 0 0],[0 0 1 1 0]);disp('Weights');
  "IW{1,1}(18,:)'" : Constant  Value=[-0.141522913770345315498389027197845280170440673828125;-0.900736196961219537371334808995015919208526611328125;-0.535519708076414691078070973162539303302764892578125;0.4771208432212954431150819800677709281444549560546875;0.21960364767590956347476094379089772701263427734375]
      mask Display: e = 0.06;c1 = [120 150 230]/255;c2 = ([120 150 230]+0)/383;c3 = ([120 150 230]+128)/383;patch([0 1 1 0],[0 0 1 1],c1);patch([0 1 1 1-e 1-e 0+e],[0 0 1 1-e 0+e 0+e],c2);patch([0 0 1 1-e 0+e 0+e],[0 1 1 1-e 1-e 0+e],c3);plot([0 1 1 0 0],[0 0 1 1 0]);disp('Weights');
  "IW{1,1}(19,:)'" : Constant  Value=[-0.331341160755560526496310558286495506763458251953125;-0.8177996491738921402969708651653490960597991943359375;-0.9527350666835499026774414232932031154632568359375;0.6102248414139079812912314082495868206024169921875;-0.6662185546675083447354381860350258648395538330078125]
      mask Display: e = 0.06;c1 = [120 150 230]/255;c2 = ([120 150 230]+0)/383;c3 = ([120 150 230]+128)/383;patch([0 1 1 0],[0 0 1 1],c1);patch([0 1 1 1-e 1-e 0+e],[0 0 1 1-e 0+e 0+e],c2);patch([0 0 1 1-e 0+e 0+e],[0 1 1 1-e 1-e 0+e],c3);plot([0 1 1 0 0],[0 0 1 1 0]);disp('Weights');
  "IW{1,1}(2,:)'" : Constant  Value=[-0.6098569334314782874884031116380356252193450927734375;-0.07302150447551358780629016109742224216461181640625;0.278647524398712764792662710533477365970611572265625;-0.9132190568660936147438178522861562669277191162109375;0.1650370493360602264232284142053686082363128662109375]
      mask Display: e = 0.06;c1 = [120 150 230]/255;c2 = ([120 150 230]+0)/383;c3 = ([120 150 230]+128)/383;patch([0 1 1 0],[0 0 1 1],c1);patch([0 1 1 1-e 1-e 0+e],[0 0 1 1-e 0+e 0+e],c2);patch([0 0 1 1-e 0+e 0+e],[0 1 1 1-e 1-e 0+e],c3);plot([0 1 1 0 0],[0 0 1 1 0]);disp('Weights');
  "IW{1,1}(20,:)'" : Constant  Value=[0.18711398838985637826937136196647770702838897705078125;0.18189384238760630818632080263341777026653289794921875;0.2059395582856118622760988046138663776218891143798828125;-0.8590102334988365395673781677032820880413055419921875;-0.6219729719119799771220868933596648275852203369140625]
      mask Display: e = 0.06;c1 = [120 150 230]/255;c2 = ([120 150 230]+0)/383;c3 = ([120 150 230]+128)/383;patch([0 1 1 0],[0 0 1 1],c1);patch([0 1 1 1-e 1-e 0+e],[0 0 1 1-e 0+e 0+e],c2);patch([0 0 1 1-e 0+e 0+e],[0 1 1 1-e 1-e 0+e],c3);plot([0 1 1 0 0],[0 0 1 1 0]);disp('Weights');
  "IW{1,1}(21,:)'" : Constant  Value=[0.78063771194357034488575663999654352664947509765625;-0.5411757951315097070477122542797587811946868896484375;-0.79020580743350732344509879112592898309230804443359375;0.8790592765790956608640271952026523649692535400390625;-0.82621363334695263613838278615730814635753631591796875]
      mask Display: e = 0.06;c1 = [120 150 230]/255;c2 = ([120 150 230]+0)/383;c3 = ([120 150 230]+128)/383;patch([0 1 1 0],[0 0 1 1],c1);patch([0 1 1 1-e 1-e 0+e],[0 0 1 1-e 0+e 0+e],c2);patch([0 0 1 1-e 0+e 0+e],[0 1 1 1-e 1-e 0+e],c3);plot([0 1 1 0 0],[0 0 1 1 0]);disp('Weights');
  "IW{1,1}(22,:)'" : Constant  Value=[0.40116755431965678280192832971806637942790985107421875;0.67977285954459254480042318391497246921062469482421875;-0.1802456661529309445146651569302775897085666656494140625;-0.01220345608326919677188993063055022503249347209930419921875;-0.357420953135742458517398745243554003536701202392578125]
      mask Display: e = 0.06;c1 = [120 150 230]/255;c2 = ([120 150 230]+0)/383;c3 = ([120 150 230]+128)/383;patch([0 1 1 0],[0 0 1 1],c1);patch([0 1 1 1-e 1-e 0+e],[0 0 1 1-e 0+e 0+e],c2);patch([0 0 1 1-e 0+e 0+e],[0 1 1 1-e 1-e 0+e],c3);plot([0 1 1 0 0],[0 0 1 1 0]);disp('Weights');
  "IW{1,1}(23,:)'" : Constant  Value=[-0.229135495394028387838858407121733762323856353759765625;0.73037982864545358818730846905964426696300506591796875;0.77634317159425580978648895325022749602794647216796875;0.51976875930445276541291832472779788076877593994140625;0.54312176585579108323287300663650967180728912353515625]
      mask Display: e = 0.06;c1 = [120 150 230]/255;c2 = ([120 150 230]+0)/383;c3 = ([120 150 230]+128)/383;patch([0 1 1 0],[0 0 1 1],c1);patch([0 1 1 1-e 1-e 0+e],[0 0 1 1-e 0+e 0+e],c2);patch([0 0 1 1-e 0+e 0+e],[0 1 1 1-e 1-e 0+e],c3);plot([0 1 1 0 0],[0 0 1 1 0]);disp('Weights');
  "IW{1,1}(24,:)'" : Constant  Value=[0.46519808169304532885490743865375407040119171142578125;0.92251063273572586620474567098426632583141326904296875;0.09226936784862767304549180380490724928677082061767578125;0.4828052898102874745944745882297866046428680419921875;-0.53341381294911205390718578200903721153736114501953125]
      mask Display: e = 0.06;c1 = [120 150 230]/255;c2 = ([120 150 230]+0)/383;c3 = ([120 150 230]+128)/383;patch([0 1 1 0],[0 0 1 1],c1);patch([0 1 1 1-e 1-e 0+e],[0 0 1 1-e 0+e 0+e],c2);patch([0 0 1 1-e 0+e 0+e],[0 1 1 1-e 1-e 0+e],c3);plot([0 1 1 0 0],[0 0 1 1 0]);disp('Weights');
  "IW{1,1}(25,:)'" : Constant  Value=[0.91375241773508519838031816107104532420635223388671875;-0.0166535828861342667661649130650403094477951526641845703125;-0.260669522276755827316918612268636934459209442138671875;0.6602212040756507693828325500362552702426910400390625;0.47835975595973934115789916177163831889629364013671875]
      mask Display: e = 0.06;c1 = [120 150 230]/255;c2 = ([120 150 230]+0)/383;c3 = ([120 150 230]+128)/383;patch([0 1 1 0],[0 0 1 1],c1);patch([0 1 1 1-e 1-e 0+e],[0 0 1 1-e 0+e 0+e],c2);patch([0 0 1 1-e 0+e 0+e],[0 1 1 1-e 1-e 0+e],c3);plot([0 1 1 0 0],[0 0 1 1 0]);disp('Weights');
  "IW{1,1}(26,:)'" : Constant  Value=[0.0856262262071023627640897757373750209808349609375;-0.5593797988627340345146876643411815166473388671875;-0.5833080343733063610756062189466319978237152099609375;-0.68699630649959697592521479236893355846405029296875;0.38563682766345852570566421491093933582305908203125]
      mask Display: e = 0.06;c1 = [120 150 230]/255;c2 = ([120 150 230]+0)/383;c3 = ([120 150 230]+128)/383;patch([0 1 1 0],[0 0 1 1],c1);patch([0 1 1 1-e 1-e 0+e],[0 0 1 1-e 0+e 0+e],c2);patch([0 0 1 1-e 0+e 0+e],[0 1 1 1-e 1-e 0+e],c3);plot([0 1 1 0 0],[0 0 1 1 0]);disp('Weights');
  "IW{1,1}(27,:)'" : Constant  Value=[0.0802116647187316456069083869806490838527679443359375;-0.5475827183174282186683967665885575115680694580078125;-0.118113446951352951685976222506724298000335693359375;-0.08538255889718282531930526602081954479217529296875;0.6481564267327606376767334950272925198078155517578125]
      mask Display: e = 0.06;c1 = [120 150 230]/255;c2 = ([120 150 230]+0)/383;c3 = ([120 150 230]+128)/383;patch([0 1 1 0],[0 0 1 1],c1);patch([0 1 1 1-e 1-e 0+e],[0 0 1 1-e 0+e 0+e],c2);patch([0 0 1 1-e 0+e 0+e],[0 1 1 1-e 1-e 0+e],c3);plot([0 1 1 0 0],[0 0 1 1 0]);disp('Weights');
  "IW{1,1}(28,:)'" : Constant  Value=[-0.383110735463427942715242124904762022197246551513671875;0.0682455943542198129048159671583562158048152923583984375;0.89992817099094202237807849087403155863285064697265625;0.2430575318609854151841176417292444966733455657958984375;0.65697619485794567228964524474577046930789947509765625]
      mask Display: e = 0.06;c1 = [120 150 230]/255;c2 = ([120 150 230]+0)/383;c3 = ([120 150 230]+128)/383;patch([0 1 1 0],[0 0 1 1],c1);patch([0 1 1 1-e 1-e 0+e],[0 0 1 1-e 0+e 0+e],c2);patch([0 0 1 1-e 0+e 0+e],[0 1 1 1-e 1-e 0+e],c3);plot([0 1 1 0 0],[0 0 1 1 0]);disp('Weights');
  "IW{1,1}(29,:)'" : Constant  Value=[-0.8575308561508325766453708638437092304229736328125;0.5242194184222948027951360927545465528964996337890625;-0.7519481667039136230101803448633290827274322509765625;0.8643667100941010428272193166776560246944427490234375;-0.4132641319832159876312971391598694026470184326171875]
      mask Display: e = 0.06;c1 = [120 150 230]/255;c2 = ([120 150 230]+0)/383;c3 = ([120 150 230]+128)/383;patch([0 1 1 0],[0 0 1 1],c1);patch([0 1 1 1-e 1-e 0+e],[0 0 1 1-e 0+e 0+e],c2);patch([0 0 1 1-e 0+e 0+e],[0 1 1 1-e 1-e 0+e],c3);plot([0 1 1 0 0],[0 0 1 1 0]);disp('Weights');
  "IW{1,1}(3,:)'" : Constant  Value=[-0.344935468265088973627285895418026484549045562744140625;-0.9799497409095019317959440741105936467647552490234375;0.83711262393739416243221285185427404940128326416015625;0.379102395004589698412900133916991762816905975341796875;0.1668010644662196728660319422488100826740264892578125]
      mask Display: e = 0.06;c1 = [120 150 230]/255;c2 = ([120 150 230]+0)/383;c3 = ([120 150 230]+128)/383;patch([0 1 1 0],[0 0 1 1],c1);patch([0 1 1 1-e 1-e 0+e],[0 0 1 1-e 0+e 0+e],c2);patch([0 0 1 1-e 0+e 0+e],[0 1 1 1-e 1-e 0+e],c3);plot([0 1 1 0 0],[0 0 1 1 0]);disp('Weights');
  "IW{1,1}(30,:)'" : Constant  Value=[-0.63603906566195700378330002422444522380828857421875;-0.3048656991024814022495093013276346027851104736328125;-0.058473508266086327012089896015822887420654296875;0.6701764711187025991279142544954083859920501708984375;-0.381261515154502017566073845955543220043182373046875]
      mask Display: e = 0.06;c1 = [120 150 230]/255;c2 = ([120 150 230]+0)/383;c3 = ([120 150 230]+128)/383;patch([0 1 1 0],[0 0 1 1],c1);patch([0 1 1 1-e 1-e 0+e],[0 0 1 1-e 0+e 0+e],c2);patch([0 0 1 1-e 0+e 0+e],[0 1 1 1-e 1-e 0+e],c3);plot([0 1 1 0 0],[0 0 1 1 0]);disp('Weights');
  "IW{1,1}(4,:)'" : Constant  Value=[0.7474986470709905628240221631131134927272796630859375;0.8168747497841710725197117426432669162750244140625;-0.691174242635366642417693583411164581775665283203125;0.9682990184540682943037381846806965768337249755859375;0.711945720685279948014567708014510571956634521484375]
      mask Display: e = 0.06;c1 = [120 150 230]/255;c2 = ([120 150 230]+0)/383;c3 = ([120 150 230]+128)/383;patch([0 1 1 0],[0 0 1 1],c1);patch([0 1 1 1-e 1-e 0+e],[0 0 1 1-e 0+e 0+e],c2);patch([0 0 1 1-e 0+e 0+e],[0 1 1 1-e 1-e 0+e],c3);plot([0 1 1 0 0],[0 0 1 1 0]);disp('Weights');
  "IW{1,1}(5,:)'" : Constant  Value=[-0.045507945520479327339291586440594983287155628204345703125;0.29777180271423142610132117624743841588497161865234375;0.439444360031744751804438919862150214612483978271484375;-0.404206836478634923270902845615637488663196563720703125;-0.91141534336125051840582500517484731972217559814453125]
      mask Display: e = 0.06;c1 = [120 150 230]/255;c2 = ([120 150 230]+0)/383;c3 = ([120 150 230]+128)/383;patch([0 1 1 0],[0 0 1 1],c1);patch([0 1 1 1-e 1-e 0+e],[0 0 1 1-e 0+e 0+e],c2);patch([0 0 1 1-e 0+e 0+e],[0 1 1 1-e 1-e 0+e],c3);plot([0 1 1 0 0],[0 0 1 1 0]);disp('Weights');
  "IW{1,1}(6,:)'" : Constant  Value=[-0.1920612556581178242964824676164425909519195556640625;-0.997161883595194087348545508575625717639923095703125;0.1554777523848185349919504005811177194118499755859375;-0.7324390000111538068239269705372862517833709716796875;0.770840190969606542381598046631552278995513916015625]
      mask Display: e = 0.06;c1 = [120 150 230]/255;c2 = ([120 150 230]+0)/383;c3 = ([120 150 230]+128)/383;patch([0 1 1 0],[0 0 1 1],c1);patch([0 1 1 1-e 1-e 0+e],[0 0 1 1-e 0+e 0+e],c2);patch([0 0 1 1-e 0+e 0+e],[0 1 1 1-e 1-e 0+e],c3);plot([0 1 1 0 0],[0 0 1 1 0]);disp('Weights');
  "IW{1,1}(7,:)'" : Constant  Value=[-0.6415370471531065543757677005487494170665740966796875;-0.9392294550101645267403682737494818866252899169921875;-0.133402045581762163095618234365247189998626708984375;0.3705593688253745465743804743397049605846405029296875;-0.1845383772880364592339219598216004669666290283203125]
      mask Display: e = 0.06;c1 = [120 150 230]/255;c2 = ([120 150 230]+0)/383;c3 = ([120 150 230]+128)/383;patch([0 1 1 0],[0 0 1 1],c1);patch([0 1 1 1-e 1-e 0+e],[0 0 1 1-e 0+e 0+e],c2);patch([0 0 1 1-e 0+e 0+e],[0 1 1 1-e 1-e 0+e],c3);plot([0 1 1 0 0],[0 0 1 1 0]);disp('Weights');
  "IW{1,1}(8,:)'" : Constant  Value=[0.938548144631420111494435332133434712886810302734375;-0.58236140105252420795522994012571871280670166015625;0.762325281278025901343653458752669394016265869140625;0.82443886502277319294762492063455283641815185546875;-0.9277908248682582570410204425570555031299591064453125]
      mask Display: e = 0.06;c1 = [120 150 230]/255;c2 = ([120 150 230]+0)/383;c3 = ([120 150 230]+128)/383;patch([0 1 1 0],[0 0 1 1],c1);patch([0 1 1 1-e 1-e 0+e],[0 0 1 1-e 0+e 0+e],c2);patch([0 0 1 1-e 0+e 0+e],[0 1 1 1-e 1-e 0+e],c3);plot([0 1 1 0 0],[0 0 1 1 0]);disp('Weights');
  "IW{1,1}(9,:)'" : Constant  Value=[-0.1850395657607827037960390725856996141374111175537109375;-0.09001875136182875547508075442237895913422107696533203125;-0.2138475357199618731574020102925715036690235137939453125;0.2217823038432571725042663501881179399788379669189453125;0.492335220996400868553877216982073150575160980224609375]
      mask Display: e = 0.06;c1 = [120 150 230]/255;c2 = ([120 150 230]+0)/383;c3 = ([120 150 230]+128)/383;patch([0 1 1 0],[0 0 1 1],c1);patch([0 1 1 1-e 1-e 0+e],[0 0 1 1-e 0+e 0+e],c2);patch([0 0 1 1-e 0+e 0+e],[0 1 1 1-e 1-e 0+e],c3);plot([0 1 1 0 0],[0 0 1 1 0]);disp('Weights');
  Mux : Mux  Inputs=30
      mask Display: e = 0.06;c1 = [120 150 230]/255;c2 = ([120 150 230]+0)/383;c3 = ([120 150 230]+128)/383;patch([0 1 1 0],[0 0 1 1],c1);patch([0 1 1 1-e 1-e 0+e],[0 0 1 1-e 0+e 0+e],c2);patch([0 0 1 1-e 0+e 0+e],[0 1 1 1-e 1-e 0+e],c3);plot([0 1 1 0 0],[0 0 1 1 0]);disp('Mux');
  dotprod{1..30} (30 alike) : neural/Weight Functions/dotprod
  "iz{1,1}" : Outport
      mask Display: e = 0.06;c1 = [120 230 180]/255;c2 = ([120 230 180]+0)/(256+128);c3 = ([120 230 180]+128)/(256+128);patch([0 1 1 0],[0 0 1 1],c1);patch([0 1 1 1-e 1-e 0+e],[0 0 1 1-e 0+e 0+e],c2);patch([0 0 1 1-e 0+e 0+e],[0 1 1 1-e 1-e 0+e],c3);plot([0 1 1 0 0],[0 0 1 1 0]);
  wires:
  Mux/1 -> "iz{1,1}"/1
  dotprod30/1 -> Mux/30
  "IW{1,1}(30,:)'"/1 -> dotprod30/1
  dotprod29/1 -> Mux/29
  "IW{1,1}(29,:)'"/1 -> dotprod29/1
  dotprod28/1 -> Mux/28
  "IW{1,1}(28,:)'"/1 -> dotprod28/1
  dotprod27/1 -> Mux/27
  "IW{1,1}(27,:)'"/1 -> dotprod27/1
  dotprod26/1 -> Mux/26
  "IW{1,1}(26,:)'"/1 -> dotprod26/1
  dotprod25/1 -> Mux/25
  "IW{1,1}(25,:)'"/1 -> dotprod25/1
  dotprod24/1 -> Mux/24
  "IW{1,1}(24,:)'"/1 -> dotprod24/1
  dotprod23/1 -> Mux/23
  "IW{1,1}(23,:)'"/1 -> dotprod23/1
  dotprod22/1 -> Mux/22
  "IW{1,1}(22,:)'"/1 -> dotprod22/1
  dotprod21/1 -> Mux/21
  "IW{1,1}(21,:)'"/1 -> dotprod21/1
  dotprod20/1 -> Mux/20
  "IW{1,1}(20,:)'"/1 -> dotprod20/1
  dotprod19/1 -> Mux/19
  "IW{1,1}(19,:)'"/1 -> dotprod19/1
  dotprod18/1 -> Mux/18
  "IW{1,1}(18,:)'"/1 -> dotprod18/1
  dotprod17/1 -> Mux/17
  "IW{1,1}(17,:)'"/1 -> dotprod17/1
  dotprod16/1 -> Mux/16
  "IW{1,1}(16,:)'"/1 -> dotprod16/1
  dotprod15/1 -> Mux/15
  "IW{1,1}(15,:)'"/1 -> dotprod15/1
  dotprod14/1 -> Mux/14
  "IW{1,1}(14,:)'"/1 -> dotprod14/1
  dotprod13/1 -> Mux/13
  "IW{1,1}(13,:)'"/1 -> dotprod13/1
  dotprod12/1 -> Mux/12
  "IW{1,1}(12,:)'"/1 -> dotprod12/1
  dotprod11/1 -> Mux/11
  "IW{1,1}(11,:)'"/1 -> dotprod11/1
  dotprod10/1 -> Mux/10
  "IW{1,1}(10,:)'"/1 -> dotprod10/1
  dotprod9/1 -> Mux/9
  "IW{1,1}(9,:)'"/1 -> dotprod9/1
  dotprod8/1 -> Mux/8
  "IW{1,1}(8,:)'"/1 -> dotprod8/1
  dotprod7/1 -> Mux/7
  "IW{1,1}(7,:)'"/1 -> dotprod7/1
  dotprod6/1 -> Mux/6
  "IW{1,1}(6,:)'"/1 -> dotprod6/1
  dotprod5/1 -> Mux/5
  "IW{1,1}(5,:)'"/1 -> dotprod5/1
  dotprod4/1 -> Mux/4
  "IW{1,1}(4,:)'"/1 -> dotprod4/1
  dotprod3/1 -> Mux/3
  "IW{1,1}(3,:)'"/1 -> dotprod3/1
  dotprod2/1 -> Mux/2
  "IW{1,1}(2,:)'"/1 -> dotprod2/1
  dotprod1/1 -> Mux/1
  "pd{1,1}"/1 -> dotprod30/2, dotprod29/2, dotprod28/2, dotprod27/2, dotprod26/2, dotprod25/2, dotprod24/2, dotprod23/2, dotprod22/2, dotprod21/2, dotprod20/2, dotprod19/2, dotprod18/2, dotprod17/2, dotprod16/2, dotprod15/2, dotprod14/2, dotprod13/2, dotprod12/2, dotprod11/2, dotprod10/2, dotprod9/2, dotprod8/2, dotprod7/2, dotprod6/2, dotprod5/2, dotprod4/2, dotprod3/2, dotprod2/2, dotprod1/2
  "IW{1,1}(1,:)'"/1 -> dotprod1/1

== system ACC5v_FFNN_traincgf_30_30_30_ep_50_Nor_20250704/Feed-Forward Neural Network/Layer 2/Delays 1 ==
  "p{2}" : Inport  PortDimensions=30
      mask Display: e = 0.06;c1 = [120 230 180]/255;c2 = ([120 230 180]+0)/(256+128);c3 = ([120 230 180]+128)/(256+128);patch([0 1 1 0],[0 0 1 1],c1);patch([0 1 1 1-e 1-e 0+e],[0 0 1 1-e 0+e 0+e],c2);patch([0 0 1 1-e 0+e 0+e],[0 1 1 1-e 1-e 0+e],c3);plot([0 1 1 0 0],[0 0 1 1 0]);
  mux : Mux  Inputs=1
      mask Display: e = 0.06;c1 = [120 150 230]/255;c2 = ([120 150 230]+0)/383;c3 = ([120 150 230]+128)/383;patch([0 1 1 0],[0 0 1 1],c1);patch([0 1 1 1-e 1-e 0+e],[0 0 1 1-e 0+e 0+e],c2);patch([0 0 1 1-e 0+e 0+e],[0 1 1 1-e 1-e 0+e],c3);plot([0 1 1 0 0],[0 0 1 1 0]);disp('Mux')
  "pd{2,1}" : Outport
      mask Display: e = 0.06;c1 = [120 230 180]/255;c2 = ([120 230 180]+0)/(256+128);c3 = ([120 230 180]+128)/(256+128);patch([0 1 1 0],[0 0 1 1],c1);patch([0 1 1 1-e 1-e 0+e],[0 0 1 1-e 0+e 0+e],c2);patch([0 0 1 1-e 0+e 0+e],[0 1 1 1-e 1-e 0+e],c3);plot([0 1 1 0 0],[0 0 1 1 0]);
  wires:
  mux/1 -> "pd{2,1}"/1
  "p{2}"/1 -> mux/1
